simulink model "tdpRecoveryMatch"  (R2026b)
settings: Solver=FixedStepDiscrete  StopTime=P.Tmatch-P.dt  FixedStep=P.dt
model workspace (MAT data in the model file):
  P.L = 9
  P.W = 6
  P.goalD = 0.6
  P.goalW = 2.6
  P.goalAreaL = 1
  P.goalAreaW = 3
  P.penMark = 1.5
  P.centreD = 1.5
  P.border = 1
  P.penAreaL = 2
  P.penAreaW = 5
  P.ballR = 0.07
  P.ballDecel = 0.4
  P.ballRestit = 0.5
  P.ballRobotE = 0.3
  P.robotR = 0.15
  P.vFwd = 0.25
  P.vBack = 0.12
  P.vSide = 0.15
  P.wMax = 0.785398163397
  P.Kp = 0.8
  P.Kw = 2
  P.avoidR = 0.7
  P.avoidGain = 0.6
  P.ballAvoidR = 0.35
  P.approachDist = 0.45
  P.kickRange = 0.28
  P.stepInSpeed = 0.1
  P.kickAlign = 0.349065850399
  P.behindTol = 0.523598775598
  P.kickNoise = 0.10471975512
  P.kickCooldown = 1
  P.shotSpeed = 1.8
  P.dribbleSpeed = 0.6
  P.maxKickSpeed = 2.2
  P.roleHyst = 0.4
  P.shootDist = 3
  P.defDist = 1.8
  P.nPerTeam = 4
  P.dt = 0.05
  P.Tmatch = 600
  P.restartPause = 2
  P.outPause = 1
  P.drawEvery = 4
  P.realtime = 0
  P.dirSign = [1 -1]
  P.seed = 1
  P.mode : TdpMode (value not decoded)
  P.rulesProfile : TdpRules (value not decoded)
  P.maxObservationAge = 0.5
  P.walkValidity = 0.1
  P.kickPreparation = 0.2
  P.kickTimeout = 1
  P.recoverTime = 0.5
  P.alignEnter = 0.35
  P.alignExit = 0.45
  P.searchTurnRate = 0.3
  P.fieldOfView = 6.28318530718
  P.observationDelay = 0
  P.observationNoise = 0
  P.fixedStriker = 0
  P.tapSpeed = 0.3
  P.freezeDuringPause = 1
  P.contactIterations = 256
  P.restartOpponentDistance = 0.75
  P.contactTolerance = 1e-10
  P.v1Enabled = 1
  P.v1MidlineBand = 0.15
  P.v1SupportTrail = 0.7
  P.v1SupportWidth = 0.8
  P.v1LooseRange = 1.2
  P.v1LooseSpeed = 0.35
  P.v1OpponentClearance = 0.6
  P.v1KeeperInset = 0.35
  P.v1ScreenDepth = 1.4
  P.v1CounterDepth = 0.4
  P.v1UnavailableWindow = [0  0; 0  0; 0  0; 0  0; 0  0; 0  0; 0  0; 0  0]
  P.v1BlindWindow = [0  0; 0  0; 0  0; 0  0; 0  0; 0  0; 0  0; 0  0]
  P.v1StaleWindow = [0  0; 0  0; 0  0; 0  0; 0  0; 0  0; 0  0; 0  0]
  P.v1StopWindow = [0 0]
  P.v1RecoveryWindow = [0  0; 0  0]
  P.v1FailWindow = [0  0; 0  0; 0  0; 0  0; 0  0; 0  0; 0  0; 0  0]
  P.v1AutoRecovery = 1
  P.v1RecoveryHealthySeconds = 0.5
  P.v1HealthDropWindow = [0  0; 0  0; 0  0; 0  0; 0  0; 0  0; 0  0; 0  0]
  feedback0(1).requestId = 0
  feedback0(1).status : TdpStatus (value not decoded)
  feedback0(1).stamp = 0
  feedback0(2).requestId = 0
  feedback0(2).status : TdpStatus (value not decoded)
  feedback0(2).stamp = 0
  feedback0(3).requestId = 0
  feedback0(3).status : TdpStatus (value not decoded)
  feedback0(3).stamp = 0
  feedback0(4).requestId = 0
  feedback0(4).status : TdpStatus (value not decoded)
  feedback0(4).stamp = 0
  feedback0(5).requestId = 0
  feedback0(5).status : TdpStatus (value not decoded)
  feedback0(5).stamp = 0
  feedback0(6).requestId = 0
  feedback0(6).status : TdpStatus (value not decoded)
  feedback0(6).stamp = 0
  feedback0(7).requestId = 0
  feedback0(7).status : TdpStatus (value not decoded)
  feedback0(7).stamp = 0
  feedback0(8).requestId = 0
  feedback0(8).status : TdpStatus (value not decoded)
  feedback0(8).stamp = 0
  health0(1).reason : TdpV1Reason (value not decoded)
  health0(1).ready = 1
  health0(1).stamp = 0
  health0(1).requestId = 0
  health0(1).activeId = 0
  health0(2).reason : TdpV1Reason (value not decoded)
  health0(2).ready = 1
  health0(2).stamp = 0
  health0(2).requestId = 0
  health0(2).activeId = 0
  health0(3).reason : TdpV1Reason (value not decoded)
  health0(3).ready = 1
  health0(3).stamp = 0
  health0(3).requestId = 0
  health0(3).activeId = 0
  health0(4).reason : TdpV1Reason (value not decoded)
  health0(4).ready = 1
  health0(4).stamp = 0
  health0(4).requestId = 0
  health0(4).activeId = 0
  health0(5).reason : TdpV1Reason (value not decoded)
  health0(5).ready = 1
  health0(5).stamp = 0
  health0(5).requestId = 0
  health0(5).activeId = 0
  health0(6).reason : TdpV1Reason (value not decoded)
  health0(6).ready = 1
  health0(6).stamp = 0
  health0(6).requestId = 0
  health0(6).activeId = 0
  health0(7).reason : TdpV1Reason (value not decoded)
  health0(7).ready = 1
  health0(7).stamp = 0
  health0(7).requestId = 0
  health0(7).activeId = 0
  health0(8).reason : TdpV1Reason (value not decoded)
  health0(8).ready = 1
  health0(8).stamp = 0
  health0(8).requestId = 0
  health0(8).activeId = 0
  request0(1).requestId = 0
  request0(1).kind : TdpAction (value not decoded)
  request0(1).velocity = [0 0 0]
  request0(1).target = [0 0]
  request0(1).speed = 0
  request0(1).stamp = 0
  request0(1).validUntil = 0
  request0(2).requestId = 0
  request0(2).kind : TdpAction (value not decoded)
  request0(2).velocity = [0 0 0]
  request0(2).target = [0 0]
  request0(2).speed = 0
  request0(2).stamp = 0
  request0(2).validUntil = 0
  request0(3).requestId = 0
  request0(3).kind : TdpAction (value not decoded)
  request0(3).velocity = [0 0 0]
  request0(3).target = [0 0]
  request0(3).speed = 0
  request0(3).stamp = 0
  request0(3).validUntil = 0
  request0(4).requestId = 0
  request0(4).kind : TdpAction (value not decoded)
  request0(4).velocity = [0 0 0]
  request0(4).target = [0 0]
  request0(4).speed = 0
  request0(4).stamp = 0
  request0(4).validUntil = 0
  request0(5).requestId = 0
  request0(5).kind : TdpAction (value not decoded)
  request0(5).velocity = [0 0 0]
  request0(5).target = [0 0]
  request0(5).speed = 0
  request0(5).stamp = 0
  request0(5).validUntil = 0
  request0(6).requestId = 0
  request0(6).kind : TdpAction (value not decoded)
  request0(6).velocity = [0 0 0]
  request0(6).target = [0 0]
  request0(6).speed = 0
  request0(6).stamp = 0
  request0(6).validUntil = 0
  request0(7).requestId = 0
  request0(7).kind : TdpAction (value not decoded)
  request0(7).velocity = [0 0 0]
  request0(7).target = [0 0]
  request0(7).speed = 0
  request0(7).stamp = 0
  request0(7).validUntil = 0
  request0(8).requestId = 0
  request0(8).kind : TdpAction (value not decoded)
  request0(8).velocity = [0 0 0]
  request0(8).target = [0 0]
  request0(8).speed = 0
  request0(8).stamp = 0
  request0(8).validUntil = 0
  v1Memory0.basePhase : TdpTeamPhase (value not decoded)
  v1Memory0.phase : TdpTeamPhase (value not decoded)
  v1Memory0.chaser = 0
  v1Memory0.failed = 0
  v1Memory0.recovering = 0
  v1Memory0.releaseId = 0
  v1Memory0.handledFailureId = 0
  v1Memory0.ballKnown = 0
  v1Memory0.ballSource = 0
  v1Memory0.takeover = 0
  v1Memory0.releaseStamp = 0
  v1Memory0.healthTiming = 0
  v1Memory0.healthySince = 0
  v1Memory0.lastHealthyStamp = 0
  v1Memory0.cancelPending = 0
  v1Memory0.releaseDeadline = 0
  v1Memory0.failureReason : TdpV1Reason (value not decoded)
  world0.robots(1).team = 1
  world0.robots(1).num = 1
  world0.robots(1).isGK = 1
  world0.robots(1).role : TdpRole (value not decoded)
  world0.robots(1).x = -4.2
  world0.robots(1).y = 0
  world0.robots(1).th = 0
  world0.robots(1).vxw = 0
  world0.robots(1).vyw = 0
  world0.robots(1).cool = 0
  world0.robots(2).team = 1
  world0.robots(2).num = 2
  world0.robots(2).isGK = 0
  world0.robots(2).role : TdpRole (value not decoded)
  world0.robots(2).x = -2.6
  world0.robots(2).y = 0.9
  world0.robots(2).th = 0
  world0.robots(2).vxw = 0
  world0.robots(2).vyw = 0
  world0.robots(2).cool = 0
  world0.robots(3).team = 1
  world0.robots(3).num = 3
  world0.robots(3).isGK = 0
  world0.robots(3).role : TdpRole (value not decoded)
  world0.robots(3).x = -2.6
  world0.robots(3).y = -0.9
  world0.robots(3).th = 0
  world0.robots(3).vxw = 0
  world0.robots(3).vyw = 0
  world0.robots(3).cool = 0
  world0.robots(4).team = 1
  world0.robots(4).num = 4
  world0.robots(4).isGK = 0
  world0.robots(4).role : TdpRole (value not decoded)
  world0.robots(4).x = -1
  world0.robots(4).y = 0
  world0.robots(4).th = 0
  world0.robots(4).vxw = 0
  world0.robots(4).vyw = 0
  world0.robots(4).cool = 0
  world0.robots(5).team = 2
  world0.robots(5).num = 1
  world0.robots(5).isGK = 1
  world0.robots(5).role : TdpRole (value not decoded)
  world0.robots(5).x = 4.2
  world0.robots(5).y = 0
  world0.robots(5).th = 3.14159265359
  world0.robots(5).vxw = 0
  world0.robots(5).vyw = 0
  world0.robots(5).cool = 0
  world0.robots(6).team = 2
  world0.robots(6).num = 2
  world0.robots(6).isGK = 0
  world0.robots(6).role : TdpRole (value not decoded)
  world0.robots(6).x = 2.6
  world0.robots(6).y = -0.9
  world0.robots(6).th = 3.14159265359
  world0.robots(6).vxw = 0
  world0.robots(6).vyw = 0
  world0.robots(6).cool = 0
  world0.robots(7).team = 2
  world0.robots(7).num = 3
  world0.robots(7).isGK = 0
  world0.robots(7).role : TdpRole (value not decoded)
  world0.robots(7).x = 2.6
  world0.robots(7).y = 0.9
  world0.robots(7).th = 3.14159265359
  world0.robots(7).vxw = 0
  world0.robots(7).vyw = 0
  world0.robots(7).cool = 0
  world0.robots(8).team = 2
  world0.robots(8).num = 4
  world0.robots(8).isGK = 0
  world0.robots(8).role : TdpRole (value not decoded)
  world0.robots(8).x = 1
  world0.robots(8).y = 0
  world0.robots(8).th = 3.14159265359
  world0.robots(8).vxw = 0
  world0.robots(8).vyw = 0
  world0.robots(8).cool = 0
  world0.ball.x = 0
  world0.ball.y = 0
  world0.ball.vx = 0
  world0.ball.vy = 0
  world0.referee.t = 0
  world0.referee.score = [0 0]
  world0.referee.lastTouch = 0
  world0.referee.pauseUntil = 0
  world0.referee.msg : TdpEvent (value not decoded)
  world0.referee.msgUntil = 2
  world0.referee.shots = [0 0]
  world0.referee.touchTime = [0 0]
  world0.actuator(1).seenId = 0
  world0.actuator(1).rejectedId = 0
  world0.actuator(1).active = 0
  world0.actuator(1).start = 0
  world0.actuator(1).target = [0 0]
  world0.actuator(1).speed = 0
  world0.actuator(1).feedback.requestId = 0
  world0.actuator(1).feedback.status : TdpStatus (value not decoded)
  world0.actuator(1).feedback.stamp = 0
  world0.actuator(1).executions = 0
  world0.actuator(2).seenId = 0
  world0.actuator(2).rejectedId = 0
  world0.actuator(2).active = 0
  world0.actuator(2).start = 0
  world0.actuator(2).target = [0 0]
  world0.actuator(2).speed = 0
  world0.actuator(2).feedback.requestId = 0
  world0.actuator(2).feedback.status : TdpStatus (value not decoded)
  world0.actuator(2).feedback.stamp = 0
  world0.actuator(2).executions = 0
  world0.actuator(3).seenId = 0
  world0.actuator(3).rejectedId = 0
  world0.actuator(3).active = 0
  world0.actuator(3).start = 0
  world0.actuator(3).target = [0 0]
  world0.actuator(3).speed = 0
  world0.actuator(3).feedback.requestId = 0
  world0.actuator(3).feedback.status : TdpStatus (value not decoded)
  world0.actuator(3).feedback.stamp = 0
  world0.actuator(3).executions = 0
  world0.actuator(4).seenId = 0
  world0.actuator(4).rejectedId = 0
  world0.actuator(4).active = 0
  world0.actuator(4).start = 0
  world0.actuator(4).target = [0 0]
  world0.actuator(4).speed = 0
  world0.actuator(4).feedback.requestId = 0
  world0.actuator(4).feedback.status : TdpStatus (value not decoded)
  world0.actuator(4).feedback.stamp = 0
  world0.actuator(4).executions = 0
  world0.actuator(5).seenId = 0
  world0.actuator(5).rejectedId = 0
  world0.actuator(5).active = 0
  world0.actuator(5).start = 0
  world0.actuator(5).target = [0 0]
  world0.actuator(5).speed = 0
  world0.actuator(5).feedback.requestId = 0
  world0.actuator(5).feedback.status : TdpStatus (value not decoded)
  world0.actuator(5).feedback.stamp = 0
  world0.actuator(5).executions = 0
  world0.actuator(6).seenId = 0
  world0.actuator(6).rejectedId = 0
  world0.actuator(6).active = 0
  world0.actuator(6).start = 0
  world0.actuator(6).target = [0 0]
  world0.actuator(6).speed = 0
  world0.actuator(6).feedback.requestId = 0
  world0.actuator(6).feedback.status : TdpStatus (value not decoded)
  world0.actuator(6).feedback.stamp = 0
  world0.actuator(6).executions = 0
  world0.actuator(7).seenId = 0
  world0.actuator(7).rejectedId = 0
  world0.actuator(7).active = 0
  world0.actuator(7).start = 0
  world0.actuator(7).target = [0 0]
  world0.actuator(7).speed = 0
  world0.actuator(7).feedback.requestId = 0
  world0.actuator(7).feedback.status : TdpStatus (value not decoded)
  world0.actuator(7).feedback.stamp = 0
  world0.actuator(7).executions = 0
  world0.actuator(8).seenId = 0
  world0.actuator(8).rejectedId = 0
  world0.actuator(8).active = 0
  world0.actuator(8).start = 0
  world0.actuator(8).target = [0 0]
  world0.actuator(8).speed = 0
  world0.actuator(8).feedback.requestId = 0
  world0.actuator(8).feedback.status : TdpStatus (value not decoded)
  world0.actuator(8).feedback.stamp = 0
  world0.actuator(8).executions = 0
  world0.active = [1 1 1 1 1 1 1 1]
  world0.lastCommands = [0  0  0; 0  0  0; 0  0  0; 0  0  0; 0  0  0; 0  0  0; 0  0  0; 0  0  0]
  world0.lastKick = 0
  world0.kickCount = 0
libraries: ControllerCore x8
settings Model: DataDictionary=TdpRecoveryTypes.sldd  Creator=fayne  LastModifiedBy=fayne
settings DataIOCC: SaveOutput=off  SignalLogging=off
settings DebuggingCC: AlgebraicLoopMsg=error

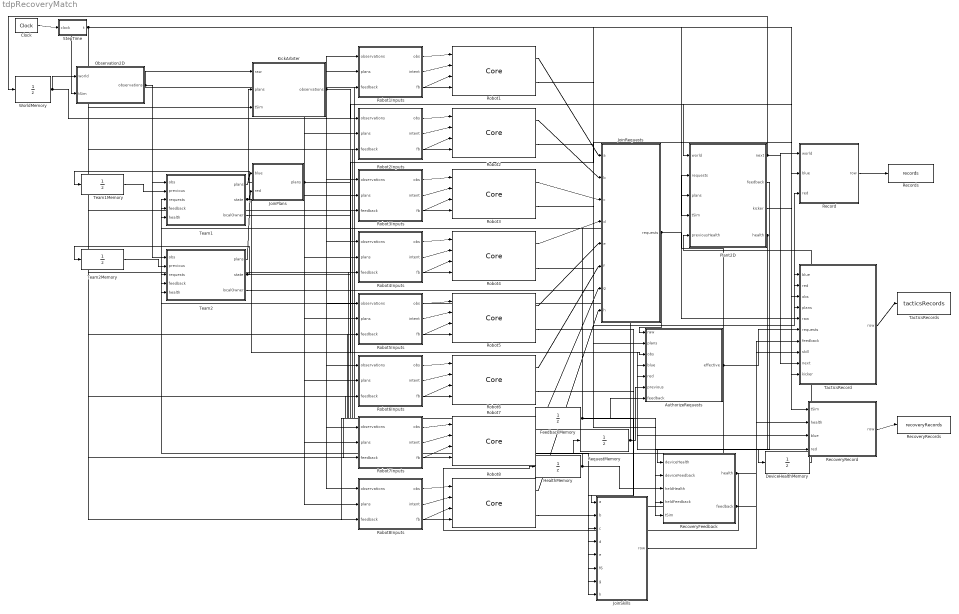
== system tdpRecoveryMatch ==
  AuthorizeRequests : MATLAB Function  TreatAsAtomicUnit=on
  Clock : DigitalClock  SampleTime=P.dt
  DeviceHealthMemory : UnitDelay  InitialCondition=health0  SampleTime=P.dt
  FeedbackMemory : UnitDelay  InitialCondition=feedback0  SampleTime=P.dt
  HealthMemory : UnitDelay  InitialCondition=health0  SampleTime=P.dt
  JoinPlans : MATLAB Function  TreatAsAtomicUnit=on
  JoinRequests : MATLAB Function  TreatAsAtomicUnit=on
  JoinSkills : MATLAB Function  TreatAsAtomicUnit=on
  KickArbiter : MATLAB Function  TreatAsAtomicUnit=on
  Observation2D : MATLAB Function  TreatAsAtomicUnit=on
  Plant2D : MATLAB Function  TreatAsAtomicUnit=on
  Record : MATLAB Function  TreatAsAtomicUnit=on
  Records : ToWorkspace  VariableName=records  SampleTime=-1
  RecoveryFeedback : MATLAB Function  TreatAsAtomicUnit=on
  RecoveryRecord : MATLAB Function  TreatAsAtomicUnit=on
  RecoveryRecords : ToWorkspace  VariableName=recoveryRecords  SampleTime=-1
  RequestMemory : UnitDelay  InitialCondition=request0  SampleTime=P.dt
  Robot{1..8} (8 alike) : ControllerCore/Core  SystemSampleTime=-1  VariantActivationTime=update diagram  EmptyChoice=off  PassThrough=off  PassThroughVariantControl=(default)  EmptyChoiceVariantControl=(default)  AllowFlexibleInterface=on  Latency=0  AutoFrameSizeCalculation=off
  Robot1Inputs : MATLAB Function  TreatAsAtomicUnit=on
  Robot2Inputs : MATLAB Function  TreatAsAtomicUnit=on
  Robot3Inputs : MATLAB Function  TreatAsAtomicUnit=on
  Robot4Inputs : MATLAB Function  TreatAsAtomicUnit=on
  Robot5Inputs : MATLAB Function  TreatAsAtomicUnit=on
  Robot6Inputs : MATLAB Function  TreatAsAtomicUnit=on
  Robot7Inputs : MATLAB Function  TreatAsAtomicUnit=on
  Robot8Inputs : MATLAB Function  TreatAsAtomicUnit=on
  StepTime : MATLAB Function  TreatAsAtomicUnit=on
  TacticsRecord : MATLAB Function  TreatAsAtomicUnit=on
  TacticsRecords : ToWorkspace  VariableName=tacticsRecords  SampleTime=-1
  Team1 : MATLAB Function  TreatAsAtomicUnit=on
  Team1Memory : UnitDelay  InitialCondition=v1Memory0  SampleTime=P.dt
  Team2 : MATLAB Function  TreatAsAtomicUnit=on
  Team2Memory : UnitDelay  InitialCondition=v1Memory0  SampleTime=P.dt
  WorldMemory : UnitDelay  InitialCondition=world0  SampleTime=P.dt
  wires:
  Clock/1 -> StepTime/1(clock)
  WorldMemory/1 -> Observation2D/1(world), Plant2D/1(world)
  StepTime/1(t) -> Observation2D/2(tSim), KickArbiter/3(tSim), Robot1/4, Robot2/4, Robot3/4, Robot4/4, Robot5/4, Robot6/4, Robot7/4, Robot8/4, RecoveryFeedback/5(tSim), Plant2D/4(tSim), RecoveryRecord/1(tSim)
  Observation2D/1(observations) -> Team1/1(obs), Team2/1(obs), KickArbiter/1(raw)
  Team1Memory/1 -> Team1/2(previous)
  RequestMemory/1 -> Team1/3(requests), Team2/3(requests), AuthorizeRequests/6(previous)
  FeedbackMemory/1 -> Team1/4(feedback), Team2/4(feedback), Robot1Inputs/3(feedback), Robot2Inputs/3(feedback), Robot3Inputs/3(feedback), Robot4Inputs/3(feedback), Robot5Inputs/3(feedback), Robot6Inputs/3(feedback), Robot7Inputs/3(feedback), Robot8Inputs/3(feedback), AuthorizeRequests/7(feedback), RecoveryFeedback/4(heldFeedback)
  HealthMemory/1 -> Team1/5(health), Team2/5(health), RecoveryFeedback/3(heldHealth)
  Team1/2(state) -> Team1Memory/1, AuthorizeRequests/4(blue), TacticsRecord/1(blue), RecoveryRecord/3(blue)
  Team2Memory/1 -> Team2/2(previous)
  Team2/2(state) -> Team2Memory/1, AuthorizeRequests/5(red), TacticsRecord/2(red), RecoveryRecord/4(red)
  Team1/1(plans) -> JoinPlans/1(blue)
  Team2/1(plans) -> JoinPlans/2(red)
  JoinPlans/1(plans) -> KickArbiter/2(plans), Robot1Inputs/2(plans), Robot2Inputs/2(plans), Robot3Inputs/2(plans), Robot4Inputs/2(plans), Robot5Inputs/2(plans), Robot6Inputs/2(plans), Robot7Inputs/2(plans), Robot8Inputs/2(plans), AuthorizeRequests/2(plans), Plant2D/3(plans), TacticsRecord/4(plans)
  KickArbiter/1(observations) -> Robot1Inputs/1(observations), Robot2Inputs/1(observations), Robot3Inputs/1(observations), Robot4Inputs/1(observations), Robot5Inputs/1(observations), Robot6Inputs/1(observations), Robot7Inputs/1(observations), Robot8Inputs/1(observations), AuthorizeRequests/3(obs), TacticsRecord/3(obs)
  Robot1Inputs/1(obs) -> Robot1/1
  Robot1Inputs/2(intent) -> Robot1/2
  Robot1Inputs/3(fb) -> Robot1/3
  Robot2Inputs/1(obs) -> Robot2/1
  Robot2Inputs/2(intent) -> Robot2/2
  Robot2Inputs/3(fb) -> Robot2/3
  Robot3Inputs/1(obs) -> Robot3/1
  Robot3Inputs/2(intent) -> Robot3/2
  Robot3Inputs/3(fb) -> Robot3/3
  Robot4Inputs/1(obs) -> Robot4/1
  Robot4Inputs/2(intent) -> Robot4/2
  Robot4Inputs/3(fb) -> Robot4/3
  Robot5Inputs/1(obs) -> Robot5/1
  Robot5Inputs/2(intent) -> Robot5/2
  Robot5Inputs/3(fb) -> Robot5/3
  Robot6Inputs/1(obs) -> Robot6/1
  Robot6Inputs/2(intent) -> Robot6/2
  Robot6Inputs/3(fb) -> Robot6/3
  Robot7Inputs/1(obs) -> Robot7/1
  Robot7Inputs/2(intent) -> Robot7/2
  Robot7Inputs/3(fb) -> Robot7/3
  Robot8Inputs/1(obs) -> Robot8/1
  Robot8Inputs/2(intent) -> Robot8/2
  Robot8Inputs/3(fb) -> Robot8/3
  Robot1/1 -> JoinRequests/1(a)
  Robot2/1 -> JoinRequests/2(b)
  Robot3/1 -> JoinRequests/3(c)
  Robot4/1 -> JoinRequests/4(d)
  Robot5/1 -> JoinRequests/5(e)
  Robot6/1 -> JoinRequests/6(f)
  Robot7/1 -> JoinRequests/7(g)
  Robot8/1 -> JoinRequests/8(h)
  JoinRequests/1(requests) -> AuthorizeRequests/1(raw), TacticsRecord/5(raw)
  AuthorizeRequests/1(effective) -> RequestMemory/1, Plant2D/2(requests), TacticsRecord/6(requests)
  Plant2D/4(health) -> RecoveryFeedback/1(deviceHealth), DeviceHealthMemory/1
  Plant2D/2(feedback) -> RecoveryFeedback/2(deviceFeedback)
  DeviceHealthMemory/1 -> Plant2D/5(previousHealth)
  RecoveryFeedback/1(health) -> HealthMemory/1, RecoveryRecord/2(health)
  Plant2D/1(next) -> WorldMemory/1, Record/1(world), TacticsRecord/9(next)
  RecoveryFeedback/2(feedback) -> FeedbackMemory/1, TacticsRecord/7(feedback)
  Team1/3(localOwner) -> Record/2(blue)
  Team2/3(localOwner) -> Record/3(red)
  Record/1(row) -> Records/1
  Robot1/2 -> JoinSkills/1(a)
  Robot2/2 -> JoinSkills/2(b)
  Robot3/2 -> JoinSkills/3(c)
  Robot4/2 -> JoinSkills/4(d)
  Robot5/2 -> JoinSkills/5(e)
  Robot6/2 -> JoinSkills/6(f6)
  Robot7/2 -> JoinSkills/7(g)
  Robot8/2 -> JoinSkills/8(h)
  JoinSkills/1(row) -> TacticsRecord/8(skill)
  Plant2D/3(kicker) -> TacticsRecord/10(kicker)
  TacticsRecord/1(row) -> TacticsRecords/1
  RecoveryRecord/1(row) -> RecoveryRecords/1

== matlab function tdpRecoveryMatch/Robot3Inputs ==
  data: observations input Bus: ObservationBus size=[1 8]; obs output Bus: ObservationBus; plans input Bus: IntentBus size=[1 8]; feedback input Bus: FeedbackBus size=[1 8]; intent output Bus: IntentBus; fb output Bus: FeedbackBus
function [obs,intent,fb]=f(observations,plans,feedback)
obs=observations(3);intent=plans(3);fb=feedback(3);
end

== matlab function tdpRecoveryMatch/Robot4Inputs ==
  data: observations input Bus: ObservationBus size=[1 8]; obs output Bus: ObservationBus; plans input Bus: IntentBus size=[1 8]; feedback input Bus: FeedbackBus size=[1 8]; intent output Bus: IntentBus; fb output Bus: FeedbackBus
function [obs,intent,fb]=f(observations,plans,feedback)
obs=observations(4);intent=plans(4);fb=feedback(4);
end

== matlab function tdpRecoveryMatch/Robot5Inputs ==
  data: observations input Bus: ObservationBus size=[1 8]; obs output Bus: ObservationBus; plans input Bus: IntentBus size=[1 8]; feedback input Bus: FeedbackBus size=[1 8]; intent output Bus: IntentBus; fb output Bus: FeedbackBus
function [obs,intent,fb]=f(observations,plans,feedback)
obs=observations(5);intent=plans(5);fb=feedback(5);
end

== matlab function tdpRecoveryMatch/Robot6Inputs ==
  data: observations input Bus: ObservationBus size=[1 8]; obs output Bus: ObservationBus; plans input Bus: IntentBus size=[1 8]; feedback input Bus: FeedbackBus size=[1 8]; intent output Bus: IntentBus; fb output Bus: FeedbackBus
function [obs,intent,fb]=f(observations,plans,feedback)
obs=observations(6);intent=plans(6);fb=feedback(6);
end

== matlab function tdpRecoveryMatch/Robot7Inputs ==
  data: observations input Bus: ObservationBus size=[1 8]; obs output Bus: ObservationBus; plans input Bus: IntentBus size=[1 8]; feedback input Bus: FeedbackBus size=[1 8]; intent output Bus: IntentBus; fb output Bus: FeedbackBus
function [obs,intent,fb]=f(observations,plans,feedback)
obs=observations(7);intent=plans(7);fb=feedback(7);
end

== matlab function tdpRecoveryMatch/Robot8Inputs ==
  data: observations input Bus: ObservationBus size=[1 8]; obs output Bus: ObservationBus; plans input Bus: IntentBus size=[1 8]; feedback input Bus: FeedbackBus size=[1 8]; intent output Bus: IntentBus; fb output Bus: FeedbackBus
function [obs,intent,fb]=f(observations,plans,feedback)
obs=observations(8);intent=plans(8);fb=feedback(8);
end

== matlab function tdpRecoveryMatch/JoinRequests ==
  data: a input Bus: RequestBus; requests output Bus: RequestBus size=[1 8]; b input Bus: RequestBus; c input Bus: RequestBus; d input Bus: RequestBus; e input Bus: RequestBus; f input Bus: RequestBus; g input Bus: RequestBus; h input Bus: RequestBus
function requests=f(a,b,c,d,e,f,g,h)
requests=[a b c d e f g h];
end

== matlab function tdpRecoveryMatch/Observation2D ==
  data: world input Bus: WorldBus; observations output Bus: ObservationBus size=[1 8]; tSim input; P parameter
function observations=f(world,tSim,P)
observations=V1Observation2D(world,tSim,P);
end

== matlab function tdpRecoveryMatch/AuthorizeRequests ==
  data: raw input Bus: RequestBus size=[1 8]; effective output Bus: RequestBus size=[1 8]; plans input Bus: IntentBus size=[1 8]; obs input Bus: ObservationBus size=[1 8]; blue input Bus: RecoveryTeamBus; red input Bus: RecoveryTeamBus; previous input Bus: RequestBus size=[1 8]; feedback input Bus: FeedbackBus size=[1 8]; P parameter
function effective=f(raw,plans,obs,blue,red,previous,feedback,P)
effective=V1AuthorizeRequests(raw,plans,obs,blue,red,previous,feedback,P);
end

== matlab function tdpRecoveryMatch/Plant2D ==
  data: world input Bus: WorldBus; next output Bus: WorldBus; requests input Bus: RequestBus size=[1 8]; plans input Bus: IntentBus size=[1 8]; tSim input; previousHealth input Bus: V1HealthBus size=[1 8]; feedback output Bus: FeedbackBus size=[1 8]; kicker output; health output Bus: V1HealthBus size=[1 8]; P parameter
function [next,feedback,kicker,health]=f(world,requests,plans,tSim,previousHealth,P)
[next,feedback,kicker,health]=RecoveryPlant2D(world,requests,plans,tSim,previousHealth,P);
end

== matlab function tdpRecoveryMatch/RecoveryFeedback ==
  data: deviceHealth input Bus: V1HealthBus size=[1 8]; health output Bus: V1HealthBus size=[1 8]; deviceFeedback input Bus: FeedbackBus size=[1 8]; heldHealth input Bus: V1HealthBus size=[1 8]; heldFeedback input Bus: FeedbackBus size=[1 8]; tSim input; feedback output Bus: FeedbackBus size=[1 8]; P parameter
function [health,feedback]=f(deviceHealth,deviceFeedback,heldHealth,heldFeedback,tSim,P)
[health,feedback]=RecoveryFeedback2D(deviceHealth,deviceFeedback,heldHealth,heldFeedback,tSim,P);
end

== matlab function tdpRecoveryMatch/Record ==
  data: world input Bus: WorldBus; row output; blue input; red input
function row=f(world,blue,red)
row=MatchRecord(world,blue,red);
end

== matlab function tdpRecoveryMatch/JoinSkills ==
  data: a input; row output; b input; c input; d input; e input; f6 input; g input; h input
function row=f(a,b,c,d,e,f6,g,h)
row=[double(a) double(b) double(c) double(d) double(e) double(f6) double(g) double(h)];
end

== matlab function tdpRecoveryMatch/TacticsRecord ==
  data: blue input Bus: RecoveryTeamBus; row output; red input Bus: RecoveryTeamBus; obs input Bus: ObservationBus size=[1 8]; plans input Bus: IntentBus size=[1 8]; raw input Bus: RequestBus size=[1 8]; requests input Bus: RequestBus size=[1 8]; feedback input Bus: FeedbackBus size=[1 8]; skill input; next input Bus: WorldBus; kicker input; P parameter
function row=f(blue,red,obs,plans,raw,requests,feedback,skill,next,kicker,P)
row=V1TacticsRecord(blue,red,obs,plans,raw,requests,feedback,skill,next,kicker,P);
end

== matlab function tdpRecoveryMatch/StepTime ==
  data: clock input; t output; P parameter
function t=f(clock,P)
t=round(clock/P.dt+1)*P.dt;
end

== matlab function tdpRecoveryMatch/RecoveryRecord ==
  data: tSim input; row output; health input Bus: V1HealthBus size=[1 8]; blue input Bus: RecoveryTeamBus; red input Bus: RecoveryTeamBus
function row=f(tSim,health,blue,red)
row=RecoveryRecord(tSim,health,blue,red);
end

== matlab function tdpRecoveryMatch/Team1 ==
  data: obs input Bus: ObservationBus size=[1 8]; plans output Bus: IntentBus size=[1 4]; previous input Bus: RecoveryTeamBus; requests input Bus: RequestBus size=[1 8]; feedback input Bus: FeedbackBus size=[1 8]; health input Bus: V1HealthBus size=[1 8]; state output Bus: RecoveryTeamBus; localOwner output; P parameter
function [plans,state,localOwner]=f(obs,previous,requests,feedback,health,P)
[plans,state]=tdp.v1TeamPlans(obs,1,previous,requests,feedback,false,P,health);
localOwner=0;
if state.chaser>0,localOwner=state.chaser-0;end
end

== matlab function tdpRecoveryMatch/Team2 ==
  data: obs input Bus: ObservationBus size=[1 8]; plans output Bus: IntentBus size=[1 4]; previous input Bus: RecoveryTeamBus; requests input Bus: RequestBus size=[1 8]; feedback input Bus: FeedbackBus size=[1 8]; health input Bus: V1HealthBus size=[1 8]; state output Bus: RecoveryTeamBus; localOwner output; P parameter
function [plans,state,localOwner]=f(obs,previous,requests,feedback,health,P)
[plans,state]=tdp.v1TeamPlans(obs,2,previous,requests,feedback,false,P,health);
localOwner=0;
if state.chaser>0,localOwner=state.chaser-4;end
end

== matlab function tdpRecoveryMatch/JoinPlans ==
  data: blue input Bus: IntentBus size=[1 4]; plans output Bus: IntentBus size=[1 8]; red input Bus: IntentBus size=[1 4]
function plans=f(blue,red)
plans=[blue red];
end

== matlab function tdpRecoveryMatch/KickArbiter ==
  data: raw input Bus: ObservationBus size=[1 8]; observations output Bus: ObservationBus size=[1 8]; plans input Bus: IntentBus size=[1 8]; tSim input; P parameter
function observations=f(raw,plans,tSim,P)
observations=KickArbiter2D(raw,plans,tSim,P);
end

== matlab function tdpRecoveryMatch/Robot1Inputs ==
  data: observations input Bus: ObservationBus size=[1 8]; obs output Bus: ObservationBus; plans input Bus: IntentBus size=[1 8]; feedback input Bus: FeedbackBus size=[1 8]; intent output Bus: IntentBus; fb output Bus: FeedbackBus
function [obs,intent,fb]=f(observations,plans,feedback)
obs=observations(1);intent=plans(1);fb=feedback(1);
end

== matlab function tdpRecoveryMatch/Robot2Inputs ==
  data: observations input Bus: ObservationBus size=[1 8]; obs output Bus: ObservationBus; plans input Bus: IntentBus size=[1 8]; feedback input Bus: FeedbackBus size=[1 8]; intent output Bus: IntentBus; fb output Bus: FeedbackBus
function [obs,intent,fb]=f(observations,plans,feedback)
obs=observations(2);intent=plans(2);fb=feedback(2);
end
